simulink model "pos_speed_ctl_pip"  (R2023a)
settings: configuration reference "config" (kept outside this file)
libraries: simulink x6
settings Model: DataDictionary=model_config.sldd  Creator=huangcheng  LastModifiedBy=Administrator
settings ConfigSetRef: SourceName=config

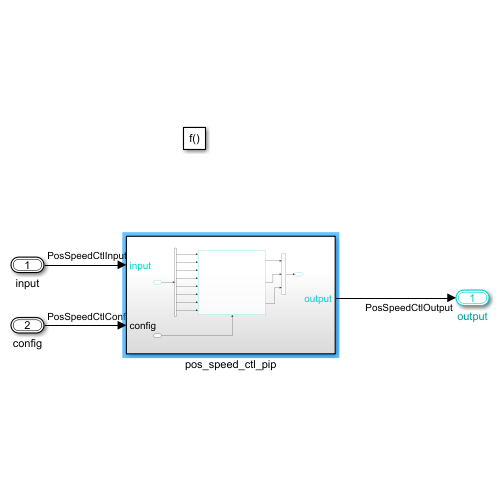
[thumbnail: Simulink's stored preview of the top-level diagram]
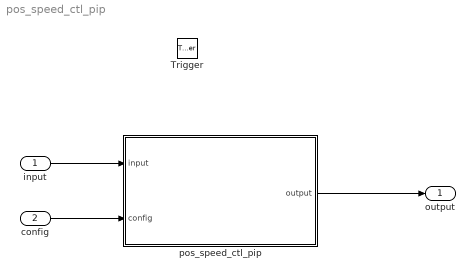
== system pos_speed_ctl_pip ==
  input : Inport  OutDataTypeStr=Bus: PosSpeedCtlInput  BusOutputAsStruct=on
  config : Inport  Port=2  OutDataTypeStr=Bus: PosSpeedCtlConfig  BusOutputAsStruct=on
  Trigger : TriggerPort  TriggerType=function-call  VariantControl=(inherit)  PortDimensions=1
  pos_speed_ctl_pip : Subsystem
  output : Outport  OutDataTypeStr=Bus: PosSpeedCtlOutput  BusOutputAsStruct=on
  wires:
  input/1 -> pos_speed_ctl_pip/1(input)
  config/1 -> pos_speed_ctl_pip/2(config)
  pos_speed_ctl_pip/1(output) -> output/1

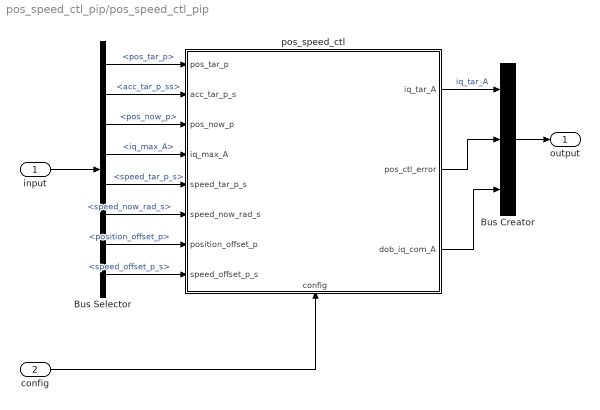
== system pos_speed_ctl_pip/pos_speed_ctl_pip ==
  input : Inport  OutDataTypeStr=Bus: PosSpeedCtlInput
  config : Inport  Port=2  OutDataTypeStr=Bus: PosSpeedCtlConfig
  Bus Creator : BusCreator  Inputs=3  OutDataTypeStr=Bus: PosSpeedCtlOutput  NonVirtualBus=on
      settings: InheritFromInputs=off
  Bus Selector : BusSelector  OutputSignals=pos_tar_p,acc_tar_p_ss,pos_now_p,iq_max_A,speed_tar_p_s,speed_now_rad_s,position_offset_p,speed_offset_p_s
  pos_speed_ctl : Subsystem
      settings: PortSchema="{\"entries\":[{\"content\":{\"sides\":[{\"content\":{\"connectorIds\":[\"In1\",\"In2\",\"In3\",\"In4\",\"In5\",\"In6\",\"In7\",\"In8\"]},\"type\":\"ConnectorPlacement.EquallySpacedRectSide\",\"uuid\":\"f3b2623c-0fa4-4d42-8778-fceddfdf52e0\"},{\"content\":{\"connectorIds\":[\"Out1\",\"Out2\",\"Out3\"],\"side\":\"RIGHT\"},\"type\":\"ConnectorPlacement.EquallySpacedRectSide\",\"uuid\":\"4dd9ec6e-ab6c-4fc9-93bd-4043d533a7d4\"},{\"content\":{\"side\":\"TOP\"},\"type\":\"ConnectorPlacement.EquallySpacedRectSide\",\"uuid\":\"d862406c-ea89-42ca-b87e-1589296646ad\"},{\"content\":{\"connectorIds\":[\"In9\"],\"side\":\"BOTTOM\"},\"type\":\"ConnectorPlacement.EquallySpacedRectSide\",\"uuid\":\"1a94dc59-2a95-4eea-bb0d-93edcb20504f\"}]},\"type\":\"ConnectorPlacement.EquallySpacedConnector\",\"uuid\":\"fd0e2535-5b2d-4b62-bdd8-8499bf5adb6e\"}],\"packageUris\":[\"http://schema.mathworks.com/mf0/Connector/R2020b\"],\"version\":\"1.0\"}"
  output : Outport  OutDataTypeStr=Bus: PosSpeedCtlOutput
  wires:
  input/1 -> Bus Selector/1
  Bus Selector/1 -> pos_speed_ctl/1(pos_tar_p)  "<pos_tar_p>"
  Bus Selector/5 -> pos_speed_ctl/5(speed_tar_p_s)  "<speed_tar_p_s>"
  Bus Selector/3 -> pos_speed_ctl/3(pos_now_p)  "<pos_now_p>"
  Bus Selector/2 -> pos_speed_ctl/2(acc_tar_p_s)  "<acc_tar_p_ss>"
  config/1 -> pos_speed_ctl/9(config)
  Bus Selector/4 -> pos_speed_ctl/4(iq_max_A)  "<iq_max_A>"
  Bus Selector/6 -> pos_speed_ctl/6(speed_now_rad_s)  "<speed_now_rad_s>"
  pos_speed_ctl/1(iq_tar_A) -> Bus Creator/1  "iq_tar_A"
  pos_speed_ctl/2(pos_ctl_error) -> Bus Creator/2
  Bus Creator/1 -> output/1
  pos_speed_ctl/3(dob_iq_com_A) -> Bus Creator/3
  Bus Selector/7 -> pos_speed_ctl/7(position_offset_p)  "<position_offset_p>"
  Bus Selector/8 -> pos_speed_ctl/8(speed_offset_p_s)  "<speed_offset_p_s>"

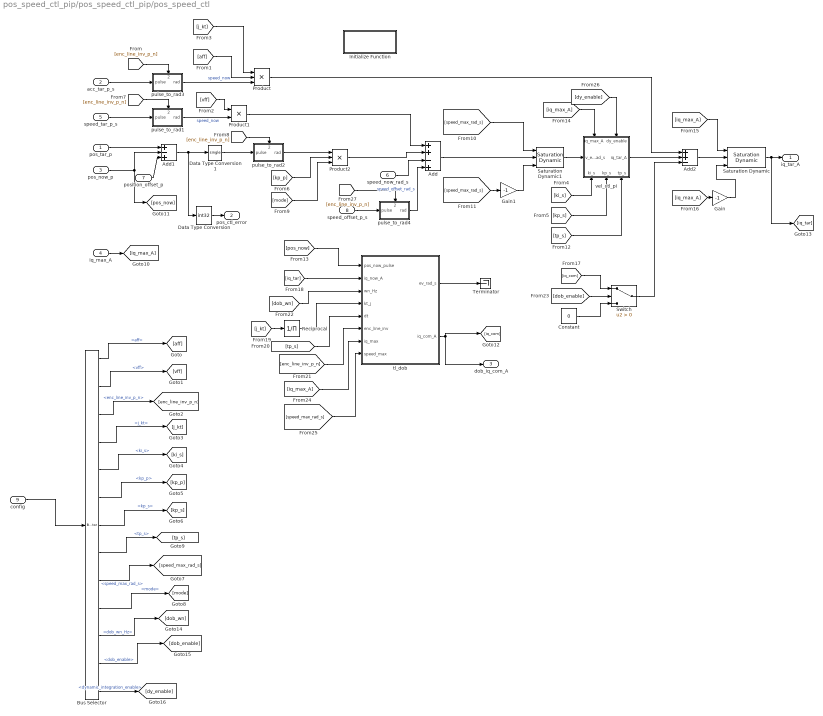
== system pos_speed_ctl_pip/pos_speed_ctl_pip/pos_speed_ctl ==
  pos_tar_p : Inport  OutDataTypeStr=int64
  acc_tar_p_s : Inport  Port=2  OutDataTypeStr=single
  pos_now_p : Inport  Port=3  OutDataTypeStr=int64
  iq_max_A : Inport  Port=4  OutDataTypeStr=single
  speed_tar_p_s : Inport  Port=5  OutDataTypeStr=single
  speed_now_rad_s : Inport  Port=6
  position_offset_p : Inport  Port=7
  speed_offset_p_s : Inport  Port=8
  config : Inport  Port=9
  Add : Sum  Inputs=++-+
  Add1 : Sum  Inputs=+-+
  Add2 : Sum  Inputs=++-
  Bus Selector : BusSelector  OutputSignals=aff,vff,enc_line_inv_p_n,j_kt,ki_s,kp_p,kp_s,tp_s,speed_max_rad_s,mode,dob_wn_Hz,dob_enable,dynamic_integration_enable
  Constant : Constant  Value=0  OutDataTypeStr=single  SampleTime=-1
  Data Type Conversion : DataTypeConversion  OutDataTypeStr=int32  SaturateOnIntegerOverflow=off  RndMeth=Floor
  Data Type Conversion1 : DataTypeConversion  OutDataTypeStr=single  SaturateOnIntegerOverflow=off  RndMeth=Floor
  Gain : Gain  Gain=-1
  Gain1 : Gain  Gain=-1
  Initialize Function : Subsystem  TreatAsAtomicUnit=on
  Product : Product  Inputs=3
  Product1 : Product
  Product2 : Product  Inputs=3
  Reciprocal : Product  Inputs=/
  Saturation Dynamic : simulink/Discontinuities/Saturation Dynamic  OutMin=[]  OutMax=[]  OutDataTypeStr=Inherit: Same as second input  OutDataType=fixdt(1, 16)  OutScaling=2^-10  DoSatur=off
  Saturation Dynamic1 : simulink/Discontinuities/Saturation Dynamic  OutMin=[]  OutMax=[]  OutDataTypeStr=Inherit: Same as second input  OutDataType=fixdt(1, 16)  OutScaling=2^-10  DoSatur=off
  Switch : Switch  Criteria=u2 > Threshold  SaturateOnIntegerOverflow=off  InputSameDT=off
  Terminator : Terminator
  pulse_to_rad1 : Subsystem
      settings: PortSchema="{\"entries\":[{\"content\":{\"sides\":[{\"content\":{\"connectorIds\":[\"In1\"]},\"type\":\"ConnectorPlacement.EquallySpacedRectSide\",\"uuid\":\"b4823d95-7c69-4874-b59f-7c369b0996d8\"},{\"content\":{\"connectorIds\":[\"Out1\"],\"side\":\"RIGHT\"},\"type\":\"ConnectorPlacement.EquallySpacedRectSide\",\"uuid\":\"88ca7b05-7b7a-41ee-b921-df5a41d5bc09\"},{\"content\":{\"connectorIds\":[\"In2\"],\"side\":\"TOP\"},\"type\":\"ConnectorPlacement.EquallySpacedRectSide\",\"uuid\":\"eb8dd953-0ac7-435c-b49c-a5d9a4d409fd\"}]},\"type\":\"ConnectorPlacement.EquallySpacedConnector\",\"uuid\":\"c2f956bc-4785-43dd-a735-6bde8e889993\"}],\"packageUris\":[\"http://schema.mathworks.com/mf0/Connector/R2020b\"],\"version\":\"1.0\"}"
  pulse_to_rad2 : Subsystem
      settings: PortSchema="{\"entries\":[{\"content\":{\"sides\":[{\"content\":{\"connectorIds\":[\"In1\"]},\"type\":\"ConnectorPlacement.EquallySpacedRectSide\",\"uuid\":\"b4823d95-7c69-4874-b59f-7c369b0996d8\"},{\"content\":{\"connectorIds\":[\"Out1\"],\"side\":\"RIGHT\"},\"type\":\"ConnectorPlacement.EquallySpacedRectSide\",\"uuid\":\"88ca7b05-7b7a-41ee-b921-df5a41d5bc09\"},{\"content\":{\"connectorIds\":[\"In2\"],\"side\":\"TOP\"},\"type\":\"ConnectorPlacement.EquallySpacedRectSide\",\"uuid\":\"eb8dd953-0ac7-435c-b49c-a5d9a4d409fd\"}]},\"type\":\"ConnectorPlacement.EquallySpacedConnector\",\"uuid\":\"c2f956bc-4785-43dd-a735-6bde8e889993\"}],\"packageUris\":[\"http://schema.mathworks.com/mf0/Connector/R2020b\"],\"version\":\"1.0\"}"
  pulse_to_rad3 : Subsystem
      settings: PortSchema="{\"entries\":[{\"content\":{\"sides\":[{\"content\":{\"connectorIds\":[\"In1\"]},\"type\":\"ConnectorPlacement.EquallySpacedRectSide\",\"uuid\":\"b4823d95-7c69-4874-b59f-7c369b0996d8\"},{\"content\":{\"connectorIds\":[\"Out1\"],\"side\":\"RIGHT\"},\"type\":\"ConnectorPlacement.EquallySpacedRectSide\",\"uuid\":\"88ca7b05-7b7a-41ee-b921-df5a41d5bc09\"},{\"content\":{\"connectorIds\":[\"In2\"],\"side\":\"TOP\"},\"type\":\"ConnectorPlacement.EquallySpacedRectSide\",\"uuid\":\"eb8dd953-0ac7-435c-b49c-a5d9a4d409fd\"}]},\"type\":\"ConnectorPlacement.EquallySpacedConnector\",\"uuid\":\"c2f956bc-4785-43dd-a735-6bde8e889993\"}],\"packageUris\":[\"http://schema.mathworks.com/mf0/Connector/R2020b\"],\"version\":\"1.0\"}"
  pulse_to_rad4 : Subsystem
      settings: PortSchema="{\"entries\":[{\"content\":{\"sides\":[{\"content\":{\"connectorIds\":[\"In1\"]},\"type\":\"ConnectorPlacement.EquallySpacedRectSide\",\"uuid\":\"b4823d95-7c69-4874-b59f-7c369b0996d8\"},{\"content\":{\"connectorIds\":[\"Out1\"],\"side\":\"RIGHT\"},\"type\":\"ConnectorPlacement.EquallySpacedRectSide\",\"uuid\":\"88ca7b05-7b7a-41ee-b921-df5a41d5bc09\"},{\"content\":{\"connectorIds\":[\"In2\"],\"side\":\"TOP\"},\"type\":\"ConnectorPlacement.EquallySpacedRectSide\",\"uuid\":\"eb8dd953-0ac7-435c-b49c-a5d9a4d409fd\"}]},\"type\":\"ConnectorPlacement.EquallySpacedConnector\",\"uuid\":\"c2f956bc-4785-43dd-a735-6bde8e889993\"}],\"packageUris\":[\"http://schema.mathworks.com/mf0/Connector/R2020b\"],\"version\":\"1.0\"}"
  tl_dob : Subsystem
  vel_ctl_pi : Subsystem  SystemSampleTime=10e-5
      settings: PortSchema="{\"entries\":[{\"content\":{\"sides\":[{\"content\":{\"connectorIds\":[\"In1\"]},\"type\":\"ConnectorPlacement.EquallySpacedRectSide\",\"uuid\":\"e3b022cc-c8b4-4571-a7fd-d1fcb297f0c3\"},{\"content\":{\"connectorIds\":[\"Out1\"],\"side\":\"RIGHT\"},\"type\":\"ConnectorPlacement.EquallySpacedRectSide\",\"uuid\":\"3bf6884c-77a3-4d83-b229-122405168209\"},{\"content\":{\"connectorIds\":[\"In2\",\"In3\"],\"side\":\"TOP\"},\"type\":\"ConnectorPlacement.EquallySpacedRectSide\",\"uuid\":\"bedad833-da8c-4704-88a9-2c09498e7db9\"},{\"content\":{\"connectorIds\":[\"In4\",\"In5\",\"In6\"],\"side\":\"BOTTOM\"},\"type\":\"ConnectorPlacement.EquallySpacedRectSide\",\"uuid\":\"108b63e0-1f0b-4eea-a7c2-8579076922f3\"}]},\"type\":\"ConnectorPlacement.EquallySpacedConnector\",\"uuid\":\"0f37a73d-3613-4aff-ba4a-eca5ad095df3\"}],\"packageUris\":[\"http://schema.mathworks.com/mf0/Connector/R2020b\"],\"version\":\"1.0\"}"
  iq_tar_A : Outport  OutDataTypeStr=single
  pos_ctl_error : Outport  Port=2
  dob_iq_com_A : Outport  Port=3
  wires:
  Gain/1 -> Saturation Dynamic/3
  pos_now_p/1 -> [pos_now], Add1/2
  Add/1 -> Saturation Dynamic1/2
  [iq_max_A] -> Saturation Dynamic/1
  Product/1 -> Add2/1
  speed_now_rad_s/1 -> Add/3
  Add1/1 -> Data Type Conversion/1, Data Type Conversion1/1
  pos_tar_p/1 -> Add1/1
  pulse_to_rad3/1(rad) -> Product/3  "speed_now"
  Data Type Conversion1/1 -> pulse_to_rad2/1(pulse)
  Saturation Dynamic/1 -> [iq_tar], iq_tar_A/1
  speed_tar_p_s/1 -> pulse_to_rad1/1(pulse)
  pulse_to_rad1/1(rad) -> Product1/2  "speed_now"
  Product1/1 -> Add/1
  vel_ctl_pi/1(iq_tar_A) -> Add2/2
  Add2/1 -> Saturation Dynamic/2
  Saturation Dynamic1/1 -> vel_ctl_pi/1(v_err_rad_s)
  pulse_to_rad2/1(rad) -> Product2/1
  Product2/1 -> Add/2
  config/1 -> Bus Selector/1
  Bus Selector/1 -> [aff]  "<aff>"
  Bus Selector/2 -> [vff]  "<vff>"
  Bus Selector/3 -> [enc_line_inv_p_n]  "<enc_line_inv_p_n>"
  Bus Selector/4 -> [j_kt]  "<j_kt>"
  Bus Selector/5 -> [ki_s]  "<ki_s>"
  Bus Selector/6 -> [kp_p]  "<kp_p>"
  Bus Selector/7 -> [kp_s]  "<kp_s>"
  Bus Selector/8 -> [tp_s]  "<tp_s>"
  [aff] -> Product/2
  [vff] -> Product1/1
  [j_kt] -> Product/1
  [ki_s] -> vel_ctl_pi/4(ki_s)
  [kp_s] -> vel_ctl_pi/5(kp_s)
  [enc_line_inv_p_n] -> pulse_to_rad3/2(enc_line_inv_p_s)
  acc_tar_p_s/1 -> pulse_to_rad3/1(pulse)
  [enc_line_inv_p_n] -> pulse_to_rad1/2(enc_line_inv_p_s)
  [kp_p] -> Product2/2
  [enc_line_inv_p_n] -> pulse_to_rad2/2(enc_line_inv_p_s)
  [speed_max_rad_s] -> Saturation Dynamic1/1
  [speed_max_rad_s] -> Gain1/1
  Gain1/1 -> Saturation Dynamic1/3
  [tp_s] -> vel_ctl_pi/6(tp_s)
  iq_max_A/1 -> [iq_max_A]
  [iq_max_A] -> vel_ctl_pi/2(iq_max_A)
  [iq_max_A] -> Gain/1
  Bus Selector/9 -> [speed_max_rad_s]  "<speed_max_rad_s>"
  Bus Selector/10 -> [mode]  "<mode>"
  [mode] -> Product2/3
  Data Type Conversion/1 -> pos_ctl_error/1
  tl_dob/2(iq_com_A) -> dob_iq_com_A/1, [iq_com]
  [pos_now] -> tl_dob/1(pos_now_pulse)
  Reciprocal/1 -> tl_dob/4(kt_j)
  [iq_tar] -> tl_dob/2(iq_now_A)
  tl_dob/1(ev_rad_s) -> Terminator/1
  [j_kt] -> Reciprocal/1
  [dob_wn] -> tl_dob/3(wn_Hz)
  [tp_s] -> tl_dob/5(dt)
  [enc_line_inv_p_n] -> tl_dob/6(enc_line_inv)
  Bus Selector/11 -> [dob_wn]  "<dob_wn_Hz>"
  Bus Selector/12 -> [dob_enable]  "<dob_enable>"
  [dob_enable] -> Switch/2
  [iq_com] -> Switch/1
  Constant/1 -> Switch/3
  Switch/1 -> Add2/3
  [iq_max_A] -> tl_dob/7(iq_max)
  [speed_max_rad_s] -> tl_dob/8(speed_max)
  Bus Selector/13 -> [dy_enable]  "<dynamic_integration_enable>"
  [dy_enable] -> vel_ctl_pi/3(dy_enable)
  position_offset_p/1 -> Add1/3
  [enc_line_inv_p_n] -> pulse_to_rad4/2(enc_line_inv_p_s)
  speed_offset_p_s/1 -> pulse_to_rad4/1(pulse)
  pulse_to_rad4/1(rad) -> Add/4  "speed_offset_rad_s"

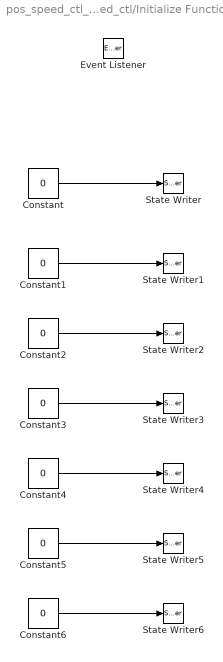
== system pos_speed_ctl_pip/pos_speed_ctl_pip/pos_speed_ctl/Initialize Function ==
  Constant{,1..2,4..6} (6 alike) : Constant  Value=0  OutDataTypeStr=single
  Constant3 : Constant  Value=0  OutDataTypeStr=int64
  Event Listener : EventListener  DisableCoverage=on  EventName=reset
  State Writer : StateWriter  StateOwnerBlock=../../vel_ctl_pi/Delay  StateName=speed_ki_int
  State Writer1 : StateWriter  StateOwnerBlock=../../vel_ctl_pi/Delay1  StateName=iq_tar_last
  State Writer2 : StateWriter  StateOwnerBlock=../../tl_dob/Delay  StateName=ev_last
  State Writer3 : StateWriter  StateOwnerBlock=../../tl_dob/Delay1  StateName=pos_now_pulse_last
  State Writer4 : StateWriter  StateOwnerBlock=../../tl_dob/dis_int/Delay3  StateName=x2_ev_rad_s
  State Writer5 : StateWriter  StateOwnerBlock=../../tl_dob/dis_int1/Delay3  StateName=x3
  State Writer6 : StateWriter  StateOwnerBlock=../../tl_dob/Delay2  StateName=x_err_last
  wires:
  Constant/1 -> State Writer/1
  Constant1/1 -> State Writer1/1
  Constant2/1 -> State Writer2/1
  Constant3/1 -> State Writer3/1
  Constant4/1 -> State Writer4/1
  Constant5/1 -> State Writer5/1
  Constant6/1 -> State Writer6/1

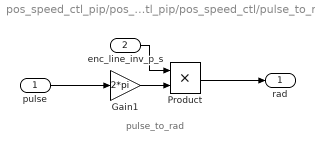
== system pos_speed_ctl_pip/pos_speed_ctl_pip/pos_speed_ctl/pulse_to_rad1 ==
  note: pulse_to_rad
  pulse : Inport
  enc_line_inv_p_s : Inport  Port=2
  Gain1 : Gain  Gain=2*pi
  Product : Product
  rad : Outport
  wires:
  enc_line_inv_p_s/1 -> Product/1
  pulse/1 -> Gain1/1
  Product/1 -> rad/1
  Gain1/1 -> Product/2

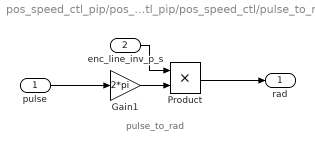
== system pos_speed_ctl_pip/pos_speed_ctl_pip/pos_speed_ctl/pulse_to_rad2 ==
  note: pulse_to_rad
  pulse : Inport
  enc_line_inv_p_s : Inport  Port=2
  Gain1 : Gain  Gain=2*pi
  Product : Product
  rad : Outport
  wires:
  Gain1/1 -> Product/2
  Product/1 -> rad/1
  pulse/1 -> Gain1/1
  enc_line_inv_p_s/1 -> Product/1

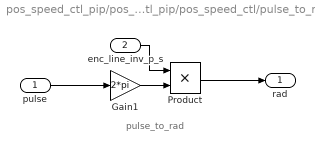
== system pos_speed_ctl_pip/pos_speed_ctl_pip/pos_speed_ctl/pulse_to_rad3 ==
  note: pulse_to_rad
  pulse : Inport
  enc_line_inv_p_s : Inport  Port=2
  Gain1 : Gain  Gain=2*pi
  Product : Product
  rad : Outport
  wires:
  Gain1/1 -> Product/2
  Product/1 -> rad/1
  pulse/1 -> Gain1/1
  enc_line_inv_p_s/1 -> Product/1

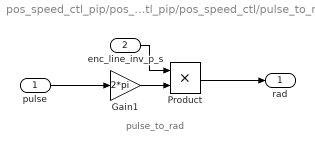
== system pos_speed_ctl_pip/pos_speed_ctl_pip/pos_speed_ctl/pulse_to_rad4 ==
  note: pulse_to_rad
  pulse : Inport
  enc_line_inv_p_s : Inport  Port=2
  Gain1 : Gain  Gain=2*pi
  Product : Product
  rad : Outport
  wires:
  enc_line_inv_p_s/1 -> Product/1
  pulse/1 -> Gain1/1
  Product/1 -> rad/1
  Gain1/1 -> Product/2

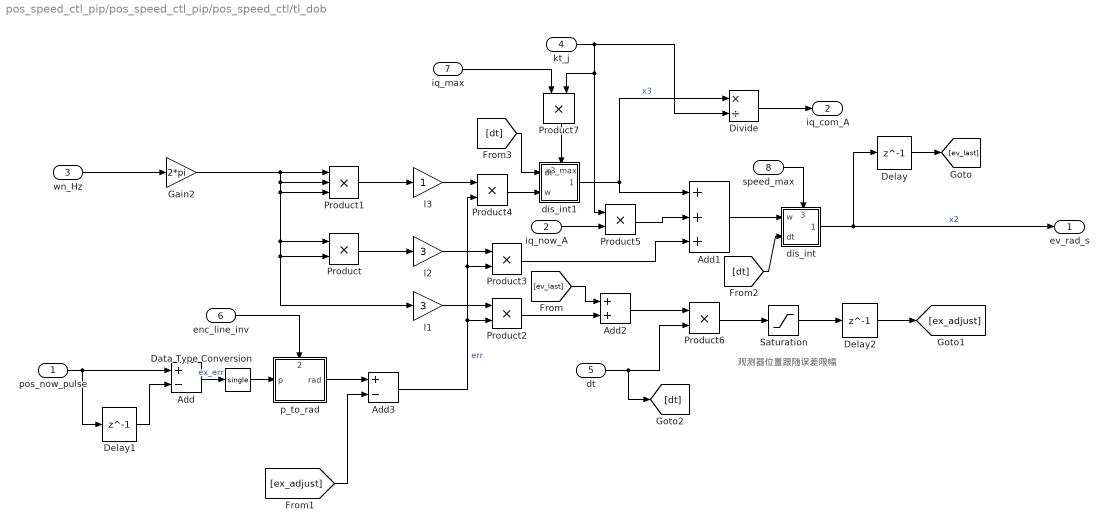
== system pos_speed_ctl_pip/pos_speed_ctl_pip/pos_speed_ctl/tl_dob ==
  note: 观测器位置跟随误差限幅
  pos_now_pulse : Inport  OutDataTypeStr=int64
  iq_now_A : Inport  Port=2
  wn_Hz : Inport  Port=3
  kt_j : Inport  Port=4
  dt : Inport  Port=5  OutDataTypeStr=single
  enc_line_inv : Inport  Port=6  OutDataTypeStr=single
  iq_max : Inport  Port=7
  speed_max : Inport  Port=8
  Add : Sum  Inputs=+-
  Add1 : Sum  Inputs=+++
  Add2 : Sum
  Add3 : Sum  Inputs=+-
  Data Type Conversion : DataTypeConversion  OutDataTypeStr=single  SaturateOnIntegerOverflow=off  RndMeth=Floor
  Delay : Delay  DelayLength=1  StateName=ev_last
  Delay1 : Delay  DelayLength=1  StateName=pos_now_pulse_last
  Delay2 : Delay  DelayLength=1  StateName=x_err_last
  Divide : Product  Inputs=*/
  Gain2 : Gain  Gain=2*pi
  Product{,2..7} (7 alike) : Product
  Product1 : Product  Inputs=3
  Saturation : Saturate  UpperLimit=pi  LowerLimit=-pi
  dis_int : Subsystem
      settings: PortSchema="{\"entries\":[{\"content\":{\"sides\":[{\"content\":{\"connectorIds\":[\"In1\",\"In2\"]},\"type\":\"ConnectorPlacement.EquallySpacedRectSide\",\"uuid\":\"d9093690-8691-44f8-9773-82e2f2723ac9\"},{\"content\":{\"connectorIds\":[\"Out1\"],\"side\":\"RIGHT\"},\"type\":\"ConnectorPlacement.EquallySpacedRectSide\",\"uuid\":\"c1202af0-84c1-4673-a3a0-1e0d634fd907\"},{\"content\":{\"connectorIds\":[\"In3\"],\"side\":\"TOP\"},\"type\":\"ConnectorPlacement.EquallySpacedRectSide\",\"uuid\":\"a27a0110-0683-4c0b-b4d0-573246df99d9\"}]},\"type\":\"ConnectorPlacement.EquallySpacedConnector\",\"uuid\":\"c8acad7b-a492-4314-bb7f-6ad97a830f2f\"}],\"packageUris\":[\"http://schema.mathworks.com/mf0/Connector/R2020b\"],\"version\":\"1.0\"}"
  dis_int1 : Subsystem
      settings: PortSchema="{\"entries\":[{\"content\":{\"sides\":[{\"content\":{\"connectorIds\":[\"In1\",\"In2\"]},\"type\":\"ConnectorPlacement.EquallySpacedRectSide\",\"uuid\":\"d9093690-8691-44f8-9773-82e2f2723ac9\"},{\"content\":{\"connectorIds\":[\"Out1\"],\"side\":\"RIGHT\"},\"type\":\"ConnectorPlacement.EquallySpacedRectSide\",\"uuid\":\"c1202af0-84c1-4673-a3a0-1e0d634fd907\"},{\"content\":{\"connectorIds\":[\"In3\"],\"side\":\"TOP\"},\"type\":\"ConnectorPlacement.EquallySpacedRectSide\",\"uuid\":\"a27a0110-0683-4c0b-b4d0-573246df99d9\"}]},\"type\":\"ConnectorPlacement.EquallySpacedConnector\",\"uuid\":\"c8acad7b-a492-4314-bb7f-6ad97a830f2f\"}],\"packageUris\":[\"http://schema.mathworks.com/mf0/Connector/R2020b\"],\"version\":\"1.0\"}"
  l1 : Gain  Gain=3
  l2 : Gain  Gain=3
  l3 : Gain
  p_to_rad : Subsystem
      settings: PortSchema="{\"entries\":[{\"content\":{\"sides\":[{\"content\":{\"connectorIds\":[\"In1\"]},\"type\":\"ConnectorPlacement.EquallySpacedRectSide\",\"uuid\":\"0fb7d365-52bb-45b4-b095-e8292e3e6273\"},{\"content\":{\"connectorIds\":[\"Out1\"],\"side\":\"RIGHT\"},\"type\":\"ConnectorPlacement.EquallySpacedRectSide\",\"uuid\":\"5a501d3d-443a-4b2d-ba2a-e55bc91f258f\"},{\"content\":{\"connectorIds\":[\"In2\"],\"side\":\"TOP\"},\"type\":\"ConnectorPlacement.EquallySpacedRectSide\",\"uuid\":\"04bb720e-b8d2-47f9-83e5-b29a4476ee16\"}]},\"type\":\"ConnectorPlacement.EquallySpacedConnector\",\"uuid\":\"b41f89c5-b036-4be3-ae65-821e33ab7d13\"}],\"packageUris\":[\"http://schema.mathworks.com/mf0/Connector/R2020b\"],\"version\":\"1.0\"}"
  ev_rad_s : Outport
  iq_com_A : Outport  Port=2
  wires:
  pos_now_pulse/1 -> Delay1/1, Add/1
  Delay1/1 -> Add/2
  Add/1 -> Data Type Conversion/1  "ex_err"
  Data Type Conversion/1 -> p_to_rad/1(p)
  Product/1 -> l2/1
  Product1/1 -> l3/1
  dis_int1/1(int) -> Divide/1, Add1/1  "x3"
  l1/1 -> Product2/1
  Product2/1 -> Add2/2
  dis_int/1(int) -> Delay/1, ev_rad_s/1  "x2"
  Delay/1 -> [ev_last]
  [ev_last] -> Add2/1
  Add2/1 -> Product6/1
  Delay2/1 -> [ex_adjust]
  p_to_rad/1(rad) -> Add3/1
  Add3/1 -> Product4/2, Product3/2, Product2/2  "err"
  [ex_adjust] -> Add3/2
  l2/1 -> Product3/1
  iq_now_A/1 -> Product5/2
  Product3/1 -> Add1/3
  Product5/1 -> Add1/2
  l3/1 -> Product4/1
  Product4/1 -> dis_int1/2(w)
  Add1/1 -> dis_int/1(w)
  wn_Hz/1 -> Gain2/1
  Product6/1 -> Saturation/1
  Gain2/1 -> Product/1, Product/2, l1/1, Product1/3, Product1/2, Product1/1
  kt_j/1 -> Product7/2, Product5/1, Divide/2
  Divide/1 -> iq_com_A/1
  dt/1 -> [dt], Product6/2
  enc_line_inv/1 -> p_to_rad/2(enc_line_inv)
  [dt] -> dis_int/2(dt)
  [dt] -> dis_int1/1(dt)
  iq_max/1 -> Product7/1
  Product7/1 -> dis_int1/3(x3_max)
  speed_max/1 -> dis_int/3(speed_max)
  Saturation/1 -> Delay2/1

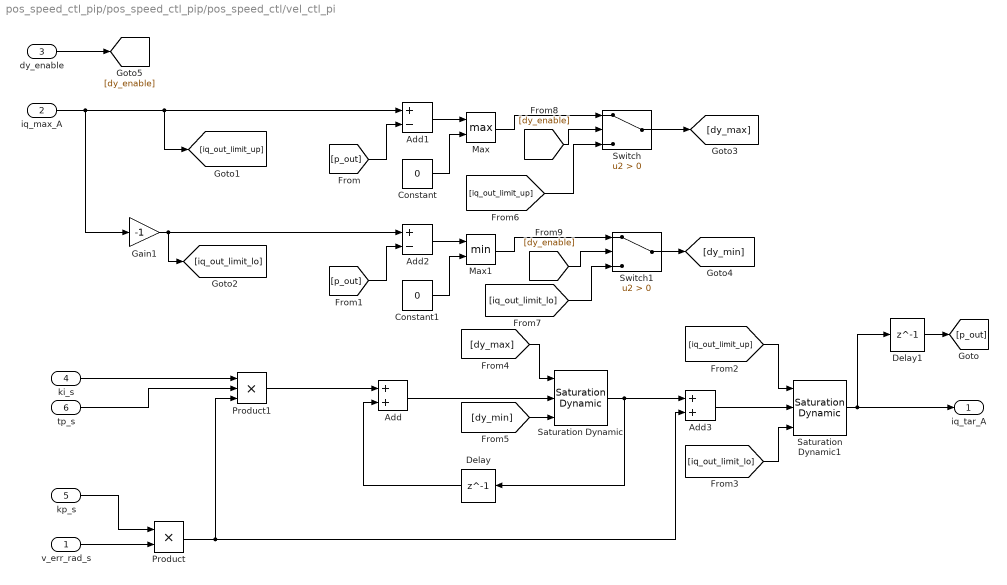
== system pos_speed_ctl_pip/pos_speed_ctl_pip/pos_speed_ctl/vel_ctl_pi ==
  v_err_rad_s : Inport
  iq_max_A : Inport  Port=2
  dy_enable : Inport  Port=3
  ki_s : Inport  Port=4
  kp_s : Inport  Port=5
  tp_s : Inport  Port=6
  Add : Sum
  Add1 : Sum  Inputs=+-
  Add2 : Sum  Inputs=+-
  Add3 : Sum
  Constant : Constant  Value=0  OutDataTypeStr=single
  Constant1 : Constant  Value=0  OutDataTypeStr=single
  Delay : Delay  DelayLength=1  StateName=speed_ki_int
  Delay1 : Delay  DelayLength=1  StateName=iq_tar_last
  Gain1 : Gain  Gain=-1
  Max : MinMax  Function=max  Inputs=2
  Max1 : MinMax  Inputs=2
  Product : Product
  Product1 : Product  Inputs=3
  Saturation Dynamic : simulink/Discontinuities/Saturation Dynamic  OutMin=[]  OutMax=[]  OutDataTypeStr=Inherit: Same as second input  OutDataType=fixdt(1, 16)  OutScaling=2^-10  DoSatur=off
  Saturation Dynamic1 : simulink/Discontinuities/Saturation Dynamic  OutMin=[]  OutMax=[]  OutDataTypeStr=Inherit: Same as second input  OutDataType=fixdt(1, 16)  OutScaling=2^-10  DoSatur=off
  Switch : Switch  Criteria=u2 > Threshold  SaturateOnIntegerOverflow=off  InputSameDT=off
  Switch1 : Switch  Criteria=u2 > Threshold  SaturateOnIntegerOverflow=off  InputSameDT=off
  iq_tar_A : Outport  OutDataTypeStr=single
  wires:
  v_err_rad_s/1 -> Product/2
  Add2/1 -> Max1/1
  [iq_out_limit_lo] -> Saturation Dynamic1/3
  [p_out] -> Add1/2
  [iq_out_limit_up] -> Saturation Dynamic1/1
  Gain1/1 -> Add2/1, [iq_out_limit_lo]
  Constant/1 -> Max/2
  [p_out] -> Add2/2
  Constant1/1 -> Max1/2
  Add3/1 -> Saturation Dynamic1/2
  iq_max_A/1 -> Add1/1, [iq_out_limit_up], Gain1/1
  Saturation Dynamic/1 -> Delay/1, Add3/1
  Add1/1 -> Max/1
  Delay1/1 -> [p_out]
  Saturation Dynamic1/1 -> iq_tar_A/1, Delay1/1
  Product1/1 -> Add/1
  Delay/1 -> Add/2
  Add/1 -> Saturation Dynamic/2
  kp_s/1 -> Product/1
  Product/1 -> Product1/3, Add3/2
  ki_s/1 -> Product1/1
  tp_s/1 -> Product1/2
  [dy_max] -> Saturation Dynamic/1
  [dy_min] -> Saturation Dynamic/3
  Switch/1 -> [dy_max]
  Switch1/1 -> [dy_min]
  Max/1 -> Switch/1
  Max1/1 -> Switch1/1
  [iq_out_limit_up] -> Switch/3
  [iq_out_limit_lo] -> Switch1/3
  dy_enable/1 -> [dy_enable]
  [dy_enable] -> Switch/2
  [dy_enable] -> Switch1/2

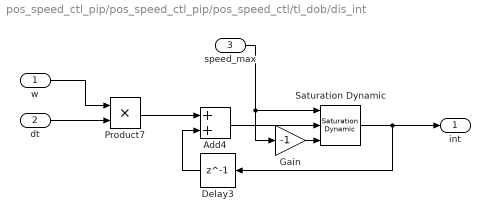
== system pos_speed_ctl_pip/pos_speed_ctl_pip/pos_speed_ctl/tl_dob/dis_int ==
  w : Inport
  dt : Inport  Port=2
  speed_max : Inport  Port=3
  Add4 : Sum
  Delay3 : Delay  DelayLength=1  StateName=x2_ev_rad_s
  Gain : Gain  Gain=-1
  Product7 : Product
  Saturation Dynamic : simulink/Discontinuities/Saturation Dynamic  OutMin=[]  OutMax=[]  OutDataTypeStr=Inherit: Same as second input  OutDataType=fixdt(1, 16)  OutScaling=2^-10  DoSatur=off
  int : Outport
  wires:
  w/1 -> Product7/1
  Delay3/1 -> Add4/2
  Product7/1 -> Add4/1
  dt/1 -> Product7/2
  Add4/1 -> Saturation Dynamic/2
  speed_max/1 -> Saturation Dynamic/1, Gain/1
  Gain/1 -> Saturation Dynamic/3
  Saturation Dynamic/1 -> Delay3/1, int/1

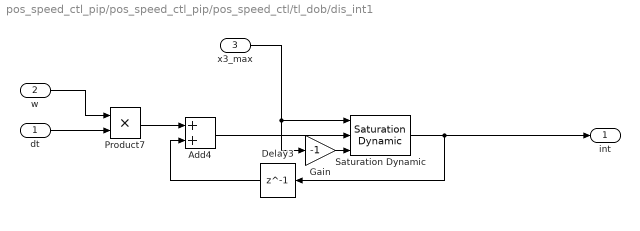
== system pos_speed_ctl_pip/pos_speed_ctl_pip/pos_speed_ctl/tl_dob/dis_int1 ==
  dt : Inport
  w : Inport  Port=2
  x3_max : Inport  Port=3
  Add4 : Sum
  Delay3 : Delay  DelayLength=1  StateName=x3
  Gain : Gain  Gain=-1
  Product7 : Product
  Saturation Dynamic : simulink/Discontinuities/Saturation Dynamic  OutMin=[]  OutMax=[]  OutDataTypeStr=Inherit: Same as second input  OutDataType=fixdt(1, 16)  OutScaling=2^-10  DoSatur=off
  int : Outport
  wires:
  w/1 -> Product7/1
  Delay3/1 -> Add4/2
  Product7/1 -> Add4/1
  dt/1 -> Product7/2
  Add4/1 -> Saturation Dynamic/2
  Saturation Dynamic/1 -> Delay3/1, int/1
  x3_max/1 -> Saturation Dynamic/1, Gain/1
  Gain/1 -> Saturation Dynamic/3

== system pos_speed_ctl_pip/pos_speed_ctl_pip/pos_speed_ctl/tl_dob/p_to_rad ==
  note: pulse_to_rad
  p : Inport
  enc_line_inv : Inport  Port=2
  Gain1 : Gain  Gain=2*pi
  Product : Product
  rad : Outport
  wires:
  p/1 -> Gain1/1
  Gain1/1 -> Product/2
  Product/1 -> rad/1
  enc_line_inv/1 -> Product/1
